simulink model "PID"  (Simulink 6.3)
settings: Solver=ode45  StartTime=0.0  StopTime=100  RelTol=1e-3
libraries: simulink_extras x1
settings Model: LastModifiedBy=33242

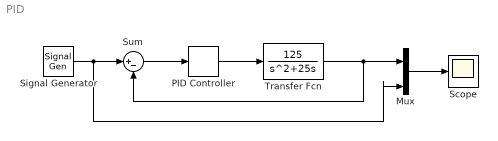
== system PID ==
  Mux : Mux  Inputs=2
  PID Controller : simulink_extras/Additional Linear/PID Controller  P=100  I=3  D=1
  Scope : Scope
  Signal Generator : SignalGenerator  Frequency=0.4*pi
  Sum : Sum  Inputs=|+-
  Transfer Fcn : TransferFcn  Numerator=[125]  Denominator=[1 25 0]
  wires:
  Signal Generator/1 -> Sum/1, Mux/2
  Sum/1 -> PID Controller/1
  PID Controller/1 -> Transfer Fcn/1
  Transfer Fcn/1 -> Sum/2, Mux/1
  Mux/1 -> Scope/1
